simulink model "Model_31_01_1"  (R2024b)
settings: Solver=ode4  StartTime=0.0  StopTime=100  FixedStep=0.01  RelTol=1e-3
values from neighbouring files (symbols this model uses):
  A_smorzata_step = A_smorzata(1:2*j_ottimo,1:2*j_ottimo)    [Code_31_01.m]
  B_smorzata_step = B_smorzata(1:2*j_ottimo,1)    [Code_31_01.m]
  C_smorzata_step = ones(1,4) * C_smorzata_step    [Code_31_01.m]
  D_smorzata_step = D_smorzata_step(1)    [Code_31_01.m]
  x0 = [0 0 0 0 0 0 0 0]'    [Code_31_01.m]    (also in ppp.m = zeros(2*j_ottimo, 1))
settings Model: Creator=baron  LastModifiedBy=baron

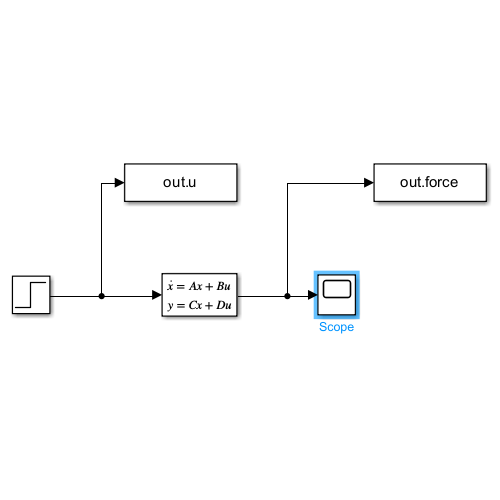
[thumbnail: Simulink's stored preview of the top-level diagram]
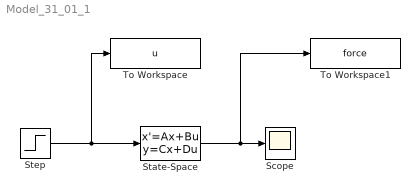
== system Model_31_01_1 ==
  Scope : Scope
  State-Space : StateSpace  A=A_smorzata_step  B=B_smorzata_step  C=C_smorzata_step  D=D_smorzata_step  InitialCondition=x0
  Step : Step  Time=0  SampleTime=0
  To Workspace : ToWorkspace  VariableName=u  SampleTime=-1
  To Workspace1 : ToWorkspace  VariableName=force  SampleTime=-1
  wires:
  Step/1 -> To Workspace/1, State-Space/1
  State-Space/1 -> To Workspace1/1, Scope/1
